simulink model "A63_SwingUp_Control"  (R2022a)
settings: Solver=FixedStepDiscrete  StartTime=0.0  StopTime=inf  FixedStep=0.000125  RelTol=1e-3  EnableMultiTasking=on
PreLoadFcn:
  | RTWConfigurationCB('preloadfcn', bdroot);c2000_ccp_data;
values from neighbouring files (symbols this model uses):
  g = 9.81    [CalcExp.m]    (also in Calculations.m; workspace.mat)
  I = m*l^2/3    (= 0.0027225)    [CalcExp.m]    (also in Calculations.m; workspace.mat)
  K = lqr(A,B,Q,R)    [CalcExp.m]    (also in Calculations.m = lqr(A,B,diag([2000 0 1000 0]),R); rscale.m = k; workspace.mat = [-31.6227766017 -20.1449549457 72.7565036852 9.8125756249])
  l = 0.165    [CalcExp.m]    (also in Calculations.m; experiments.m = P.l*opt.lScale; workspace.mat)
  m = 0.3    [CalcExp.m]    (also in Calculations.m; experiments.m = runAll(makeCtl(c, P), SC, P, opt); workspace.mat)
  Nbar = rscale(sys_ss,K)    [CalcExp.m]    (also in Calculations.m; rscale.m = Nu + K*Nx; workspace.mat = -31.6227766017)
undefined symbols (not defined in the file or in its folder): DiscIntNeverNeededParam, MaxSpeed
libraries: simulink x8, slpidlib x2, lucasnuelle x2
settings Model: SimulationMode=external  ExtModeEnableFloating=off  Creator=The MathWorks, Inc.  LastModifiedBy=Bukarov
settings SolverCC: AlgebraicLoopSolver=TrustRegion
settings DataIOCC: LimitDataPoints=on  SaveFormat=Array  SaveOutput=off  SaveTime=off  ReturnWorkspaceOutputs=off
settings OptimizationCC: DefaultParameterBehavior=Inlined  ExpressionDepthLimit=2147483647  InitFltsAndDblsToZero=on  LifeSpan=inf  MaxStackSize=64  EfficientTunableParamExpr=on
settings DebuggingCC: UnderspecifiedInitializationDetection=Classic  MergeDetectMultiDrivingBlocksExec=none  CheckExecutionContextPreStartOutputMsg=on  SignalResolutionControl=TryResolveAllWithWarning  SolverPrmCheckMsg=warning  MultiTaskDSMMsg=warning  MultiTaskCondExecSysMsg=none  SigSpecEnsureSampleTimeMsg=none  FcnCallInpInsideContextMsg=warning  UnconnectedInputMsg=warning  UnconnectedOutputMsg=warning  UnconnectedLineMsg=warning  AllowSymbolicDim=off  StateNameClashWarn=warning  SFUnexpectedBacktrackingDiag=warning  SFNoUnconditionalDefaultTransitionDiag=warning  SFExecutionAtInitializationDiag=none  SFMachineParentedDataDiag=warning  ArithmeticOperatorsInVariantConditions=warning
settings HardwareCC: ProdBitPerChar=16  ProdBitPerInt=16  ProdBitPerPointer=32  ProdLargestAtomicInteger=Integer  ProdLargestAtomicFloat=None  ProdWordSize=16  ProdHWDeviceType=Texas Instruments->C2000  TargetBitPerChar=16  TargetBitPerInt=16  TargetBitPerPointer=16  TargetLargestAtomicInteger=Integer  TargetIntDivRoundTo=Zero  TargetEndianess=LittleEndian  TargetWordSize=16  TargetHWDeviceType=Texas Instruments->C2000  ProdEqTarget=off
settings ModelReferenceCC: PropagateSignalLabelsOutOfModel=off
settings SFSimCC: SimUseLocalCustomCode=off  SimParseCustomCode=off  MATLABDynamicMemAlloc=off  CustomCodeUndefinedFunction=UseInterfaceOnly
settings RTWCC: SystemTargetFile=ert.tlc  HardwareBoard=TI Delfino F2833x  TemplateMakefile=ert_default_tmf  PostCodeGenCommand=LNPostCodeGenCommand(modelName, buildInfo);codertarget.postCodeGenHookCommand(h)  RTWUseLocalCustomCode=off  CustomInclude="\"C:\\Program Files\\LN\\MatlabToolbox\\lucasnuelle\\codelibs\""  Toolchain=Texas Instruments Code Composer Studio (C2000)  BuildConfiguration=Specify  DLArmComputeVersion=19.05
settings RTWCC: CustomSource=|
  | "C:\Program Files\LN\MatlabToolbox\lucasnuelle\codelibs\sfcn_lnc_wrapper.c"
  | "C:\Program Files\LN\MatlabToolbox\lucasnuelle\codelibs\CO36202A.c"
settings RTWCC: CustomLibrary=|
  | "C:\Program Files\LN\MatlabToolbox\lucasnuelle\codelibs\LNDacCO36202A.lib"
  | "C:\Program Files\LN\MatlabToolbox\lucasnuelle\codelibs\LNComCO36202A.lib"
  | "C:\Program Files\LN\MatlabToolbox\lucasnuelle\codelibs\LNDisplay.lib"
settings CodeAppCC: ForceParamTrailComments=on  IgnoreCustomStorageClasses=off  CustomSymbolStrType=$N$R$M  StateflowObjectComments=on  InternalIdentifier=Classic
settings ERTTargetCC: MultiwordLength=2048  ParMdlRefBuildCompliant=off  CompOptLevelCompliant=off  CPPClassGenCompliant=off  ExtModeStaticAllocSize=2048  ExtModeMexFile=TIC2000ExternalModeOpen  ExtModeIntrfLevel=Level2 - Open  InlinedParameterPlacement=NonHierarchical  ConvertIfToSwitch=off  SuppressUnreachableDefaultCases=off
settings ConfigComp: CovSaveCumulativeToWorkspaceVar=on  CovSaveSingleToWorkspaceVar=on  CovExternalEMLEnable=off  CovSFcnEnable=off

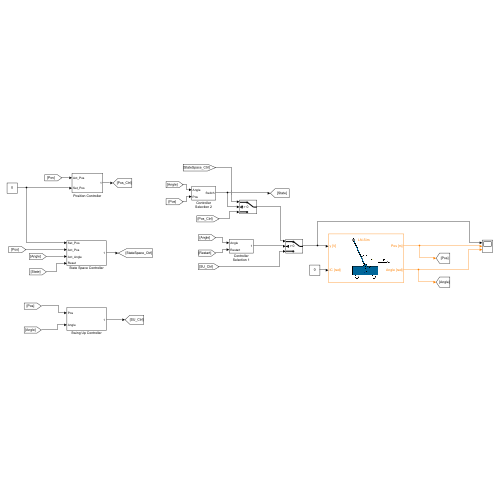
[thumbnail: Simulink's stored preview of the top-level diagram]
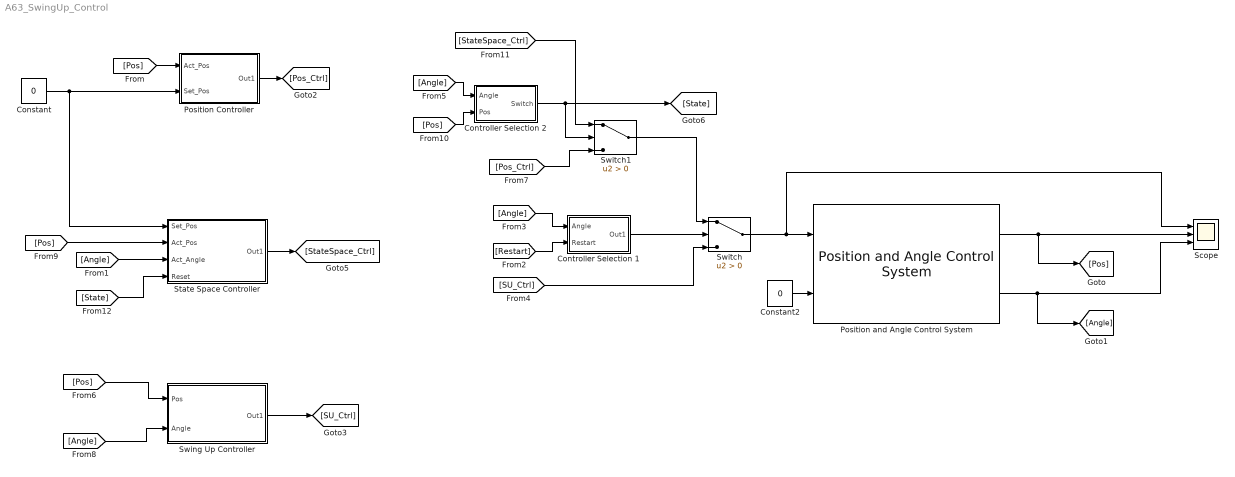
== system A63_SwingUp_Control ==
  Constant : Constant  Value=0
  Constant2 : Constant  Value=0
  Controller Selection 1 : Subsystem
  Controller Selection 2 : Subsystem
  Position Controller : Subsystem
  Position and Angle Control System : lucasnuelle/Simulation/Position and Angle Control System  DefSystem=Predefined  m=0.3  l=0.165  fr=0.3  exportData=on
      settings: SourceProductName=Lucas-Nülle
  Scope : Scope  NumInputPorts=3
  State Space Controller : Subsystem
  Swing Up Controller : Subsystem
  Switch : Switch  Criteria=u2 > Threshold  SaturateOnIntegerOverflow=off  InputSameDT=off
  Switch1 : Switch  Criteria=u2 > Threshold  SaturateOnIntegerOverflow=off  InputSameDT=off
  wires:
  [Angle] -> State Space Controller/3(Act_Angle)
  Constant/1 -> State Space Controller/1(Set_Pos), Position Controller/2(Set_Pos)
  [Pos] -> Position Controller/1(Act_Pos)
  Position Controller/1(Out1) -> [Pos_Ctrl]
  [Pos] -> State Space Controller/2(Act_Pos)
  State Space Controller/1(Out1) -> [StateSpace_Ctrl]
  [State] -> State Space Controller/4(Reset)
  [SU_Ctrl] -> Switch/3
  Controller Selection 1/1(Out1) -> Switch/2
  [Angle] -> Controller Selection 2/1(Angle)
  [Angle] -> Controller Selection 1/1(Angle)
  [Pos] -> Controller Selection 2/2(Pos)
  Switch1/1 -> Switch/1
  [StateSpace_Ctrl] -> Switch1/1
  Controller Selection 2/1(Switch) -> Switch1/2, [State]
  [Pos_Ctrl] -> Switch1/3
  [Restart] -> Controller Selection 1/2(Restart)
  Swing Up Controller/1(Out1) -> [SU_Ctrl]
  [Pos] -> Swing Up Controller/1(Pos)
  [Angle] -> Swing Up Controller/2(Angle)
  Switch/1 -> Scope/1, Position and Angle Control System/1
  Position and Angle Control System/1 -> [Pos], Scope/2
  Position and Angle Control System/2 -> Scope/3, [Angle]
  Constant2/1 -> Position and Angle Control System/2

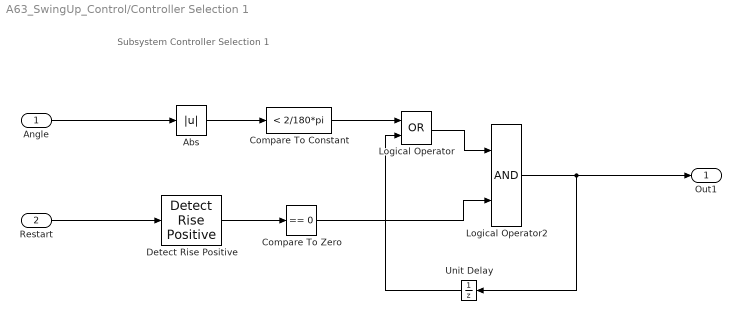
== system A63_SwingUp_Control/Controller Selection 1 ==
  note: Subsystem Controller Selection 1
  Angle : Inport
  Restart : Inport  Port=2
  Abs : Abs  SaturateOnIntegerOverflow=off
  Compare To Constant : simulink/Logic and Bit Operations/Compare To Constant  relop=<  const=2/180*pi  OutDataTypeStr=boolean
  Compare To Zero : simulink/Logic and Bit Operations/Compare To Zero  relop===  OutDataTypeStr=boolean
  Detect Rise Positive : simulink/Logic and Bit Operations/Detect Rise Positive  vinit=0  OutDataTypeStr=boolean
  Logical Operator : Logic  Operator=OR  AllPortsSameDT=off  OutDataTypeStr=boolean
  Logical Operator2 : Logic  AllPortsSameDT=off  OutDataTypeStr=boolean
  Unit Delay : UnitDelay  SampleTime=-1  HasFrameUpgradeWarning=on
  Out1 : Outport
  wires:
  Compare To Zero/1 -> Logical Operator2/2
  Detect Rise Positive/1 -> Compare To Zero/1
  Restart/1 -> Detect Rise Positive/1
  Logical Operator2/1 -> Out1/1, Unit Delay/1
  Compare To Constant/1 -> Logical Operator/1
  Logical Operator/1 -> Logical Operator2/1
  Abs/1 -> Compare To Constant/1
  Angle/1 -> Abs/1
  Unit Delay/1 -> Logical Operator/2

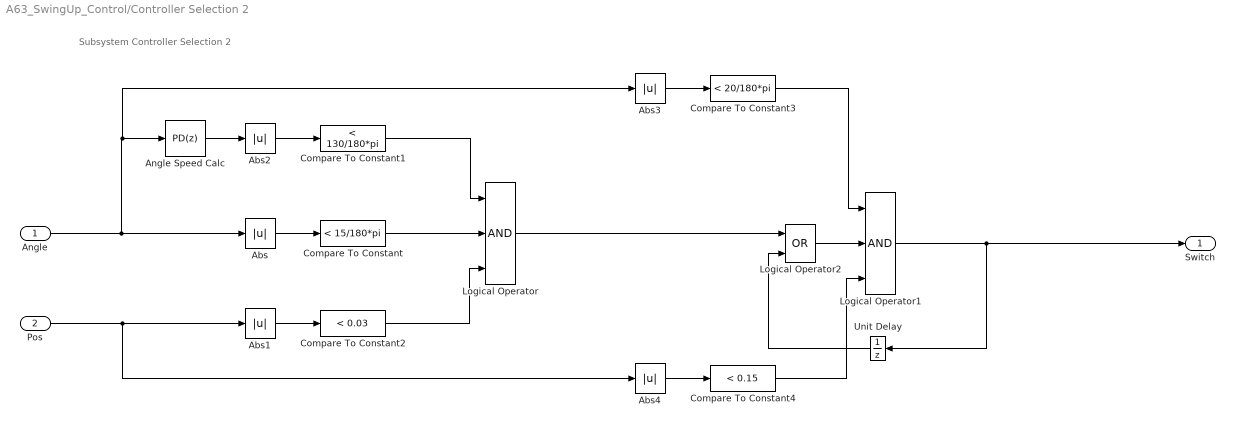
== system A63_SwingUp_Control/Controller Selection 2 ==
  note: Subsystem Controller Selection 2
  Angle : Inport
  Pos : Inport  Port=2
  Abs{,1..4} (5 alike) : Abs  SaturateOnIntegerOverflow=off
  Angle Speed Calc : slpidlib/PID Controller  Controller=PD  Form=Parallel  TimeDomain=Discrete-time  UseExternalTs=off  SampleTime=-1  IntegratorMethod=Forward Euler  FilterMethod=Forward Euler  ControllerParametersSource=internal  P=0  I=1  UseKiTs=off  D=1  N=100  UseFilter=on  TunerSelectOption=Transfer Function Based (PID Tuner App)  InitialConditionSource=internal  InitialConditionForIntegrator=0  InitialConditionForFilter=0  DifferentiatorICPrevScaledInput=0  ExternalReset=none  TrackingMode=off  Kt=1  LimitOutput=off  SatLimitsSource=internal  UpperSaturationLimit=inf  LowerSaturationLimit=-inf  LinearizeAsGain=off  AntiWindupMode=none  Kb=1  POutMin=[]  POutMax=[]  IOutMin=[]  IOutMax=[]  DOutMin=[]  DOutMax=[]  NOutMin=[]  NOutMax=[]  SumOutMin=[]  SumOutMax=[]  SaturationOutMin=[]  SaturationOutMax=[]  PParamMin=[]  PParamMax=[]  IParamMin=[]  IParamMax=[]  DParamMin=[]  DParamMax=[]  NParamMin=[]  NParamMax=[]  KbParamMin=[]  KbParamMax=[]  KtParamMin=[]  KtParamMax=[]  KbOutMin=[]  KbOutMax=[]  KtOutMin=[]  KtOutMax=[]  IntegratorOutMin=[]  IntegratorOutMax=[]  FilterOutMin=[]  FilterOutMax=[]  SumI1OutMin=[]  SumI1OutMax=[]  SumI2OutMin=[]  SumI2OutMax=[]  SumI3OutMin=[]  SumI3OutMax=[]  SumI4OutMin=[]  SumI4OutMax=[]  SumDOutMin=[]  SumDOutMax=[]  DifferentiatorOutMin=[]  DifferentiatorOutMax=[]  FilterDiffOutCoefMin=[]  FilterDiffOutCoefMax=[]  ReciprocalOutMin=[]  ReciprocalOutMax=[]  SumDenOutMin=[]  SumDenOutMax=[]  SumNumOutMin=[]  SumNumOutMax=[]  DivideOutMin=[]  DivideOutMax=[]  UdiffTsProdOutMin=[]  UdiffTsProdOutMax=[]  NTsProdOutMin=[]  NTsProdOutMax=[]  UintegralTsProdOutMin=[]  UintegralTsProdOutMax=[]  UngainTsProdOutMin=[]  UngainTsProdOutMax=[]  IntegratorContinuousStateAttributes=''  IntegratorStateMustResolveToSignalObject=off  IntegratorRTWStateStorageClass=Auto  FilterContinuousStateAttributes=''  FilterStateMustResolveToSignalObject=off  FilterRTWStateStorageClass=Auto  ParallelPVariant=InternalParameters  IdealPVariant=Disabled  IVariant=Disabled  DVariant=InternalParameters  IntegratorVariant=Disabled  SatVariant=Disabled  AWVariant=Disabled  PCopyVariant=Disabled  TRVariant=Disabled  FdbkBlocksVariant=Forward  IdealPFdbkVariant=Disabled  SatFdbkVariant=Disabled  DerivativeFilterVariant=ForwardEulerFilter  NVariant=InternalParameters  NCopyVariant=Disabled  FilterICVariant=InternalICsFilter  IntegratorICVariant=Disabled  ExternalResetVariant=Disabled  TRSumVariant=Passthrough  SumFdbkVariant=Disabled  SumVariant=Sum_PD  TsampFilterVariant=InternalTs  TsampNgainVariant=Passthrough  TsampIntegralVariant=Disabled_SignalSpec  ExternalSaturationOutDataTypeStr=Inherit: Same as second input  aMode=0
  Compare To Constant : simulink/Logic and Bit Operations/Compare To Constant  relop=<  const=15/180*pi  OutDataTypeStr=boolean
  Compare To Constant1 : simulink/Logic and Bit Operations/Compare To Constant  relop=<  const=130/180*pi  OutDataTypeStr=boolean
  Compare To Constant2 : simulink/Logic and Bit Operations/Compare To Constant  relop=<  const=0.03  OutDataTypeStr=boolean
  Compare To Constant3 : simulink/Logic and Bit Operations/Compare To Constant  relop=<  const=20/180*pi  OutDataTypeStr=boolean
  Compare To Constant4 : simulink/Logic and Bit Operations/Compare To Constant  relop=<  const=0.15  OutDataTypeStr=boolean
  Logical Operator : Logic  Inputs=3  AllPortsSameDT=off  OutDataTypeStr=boolean
  Logical Operator1 : Logic  Inputs=3  AllPortsSameDT=off  OutDataTypeStr=boolean
  Logical Operator2 : Logic  Operator=OR  AllPortsSameDT=off  OutDataTypeStr=boolean
  Unit Delay : UnitDelay  SampleTime=-1  HasFrameUpgradeWarning=on
  Switch : Outport
  wires:
  Compare To Constant4/1 -> Logical Operator1/3
  Abs4/1 -> Compare To Constant4/1
  Compare To Constant3/1 -> Logical Operator1/1
  Abs3/1 -> Compare To Constant3/1
  Angle Speed Calc/1 -> Abs2/1
  Compare To Constant1/1 -> Logical Operator/1
  Abs2/1 -> Compare To Constant1/1
  Unit Delay/1 -> Logical Operator2/2
  Logical Operator1/1 -> Switch/1, Unit Delay/1
  Logical Operator2/1 -> Logical Operator1/2
  Compare To Constant2/1 -> Logical Operator/3
  Pos/1 -> Abs1/1, Abs4/1
  Compare To Constant/1 -> Logical Operator/2
  Abs1/1 -> Compare To Constant2/1
  Angle/1 -> Angle Speed Calc/1, Abs3/1, Abs/1
  Abs/1 -> Compare To Constant/1
  Logical Operator/1 -> Logical Operator2/1

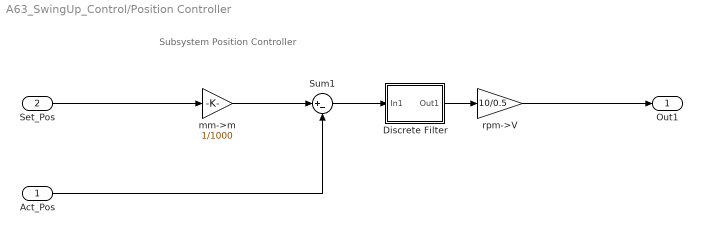
== system A63_SwingUp_Control/Position Controller ==
  note: Subsystem Position Controller
  Act_Pos : Inport
  Set_Pos : Inport  Port=2
  Discrete Filter : Subsystem
  Sum1 : Sum  Inputs=|+-
  mm->m : Gain  Gain=1/1000
  rpm->V : Gain  Gain=10/0.5
  Out1 : Outport
  wires:
  Act_Pos/1 -> Sum1/2
  mm->m/1 -> Sum1/1
  Sum1/1 -> Discrete Filter/1(In1)
  Discrete Filter/1(Out1) -> rpm->V/1
  Set_Pos/1 -> mm->m/1
  rpm->V/1 -> Out1/1

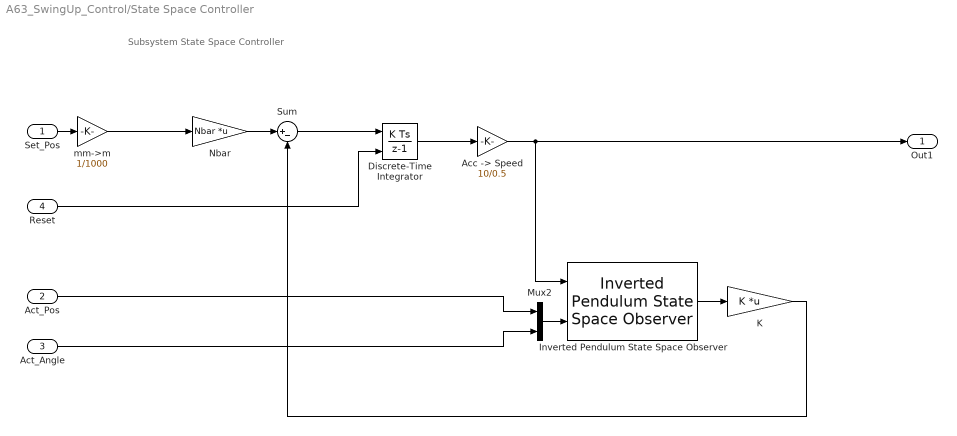
== system A63_SwingUp_Control/State Space Controller ==
  note: Subsystem State Space Controller
  Set_Pos : Inport
  Act_Pos : Inport  Port=2
  Act_Angle : Inport  Port=3
  Reset : Inport  Port=4
  "Acc -> Speed" : Gain  Gain=10/0.5
  Discrete-Time Integrator : DiscreteIntegrator  ExternalReset=rising  SampleTime=-1  ICPrevOutput=DiscIntNeverNeededParam  ICPrevScaledInput=DiscIntNeverNeededParam
  Inverted Pendulum State Space Observer : lucasnuelle/Simulation/Inverted Pendulum State Space Observer  DefSystem=Predefined  m=0.3  l=0.165  fr=0.3  exportData=on
      settings: SourceProductName=Lucas-Nülle
  K : Gain  Gain=K  Multiplication=Matrix(K*u) (u vector)
  Mux2 : Mux  Inputs=2
  Nbar : Gain  Gain=Nbar  Multiplication=Matrix(K*u) (u vector)
  Sum : Sum  Inputs=|+-
  mm->m : Gain  Gain=1/1000
  Out1 : Outport
  wires:
  mm->m/1 -> Nbar/1
  Reset/1 -> Discrete-Time Integrator/2
  Set_Pos/1 -> mm->m/1
  Discrete-Time Integrator/1 -> "Acc -> Speed"/1
  Inverted Pendulum State Space Observer/1 -> K/1
  Nbar/1 -> Sum/1
  Act_Angle/1 -> Mux2/2
  Mux2/1 -> Inverted Pendulum State Space Observer/2
  Sum/1 -> Discrete-Time Integrator/1
  Act_Pos/1 -> Mux2/1
  K/1 -> Sum/2
  "Acc -> Speed"/1 -> Out1/1, Inverted Pendulum State Space Observer/1

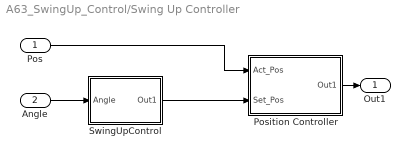
== system A63_SwingUp_Control/Swing Up Controller ==
  Pos : Inport
  Angle : Inport  Port=2
  Position Controller : Subsystem
  SwingUpControl : Subsystem
  Out1 : Outport
  wires:
  Angle/1 -> SwingUpControl/1(Angle)
  Position Controller/1(Out1) -> Out1/1
  SwingUpControl/1(Out1) -> Position Controller/2(Set_Pos)
  Pos/1 -> Position Controller/1(Act_Pos)

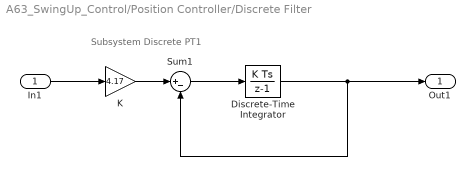
== system A63_SwingUp_Control/Position Controller/Discrete Filter ==
  note: Subsystem Discrete PT1
  In1 : Inport
  Discrete-Time Integrator : DiscreteIntegrator  gainval=1/0.17  SampleTime=-1  ICPrevOutput=DiscIntNeverNeededParam  ICPrevScaledInput=DiscIntNeverNeededParam
  K : Gain  Gain=4.17
  Sum1 : Sum  Inputs=|+-
  Out1 : Outport
  wires:
  Discrete-Time Integrator/1 -> Sum1/2, Out1/1
  K/1 -> Sum1/1
  In1/1 -> K/1
  Sum1/1 -> Discrete-Time Integrator/1

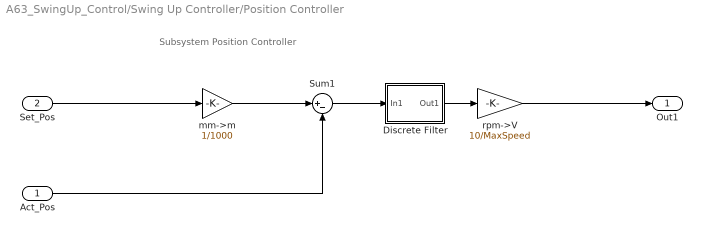
== system A63_SwingUp_Control/Swing Up Controller/Position Controller ==
  note: Subsystem Position Controller
  Act_Pos : Inport
  Set_Pos : Inport  Port=2
  Discrete Filter : Subsystem
  Sum1 : Sum  Inputs=|+-
  mm->m : Gain  Gain=1/1000
  rpm->V : Gain  Gain=10/MaxSpeed
  Out1 : Outport
  wires:
  Act_Pos/1 -> Sum1/2
  mm->m/1 -> Sum1/1
  Sum1/1 -> Discrete Filter/1(In1)
  Discrete Filter/1(Out1) -> rpm->V/1
  Set_Pos/1 -> mm->m/1
  rpm->V/1 -> Out1/1

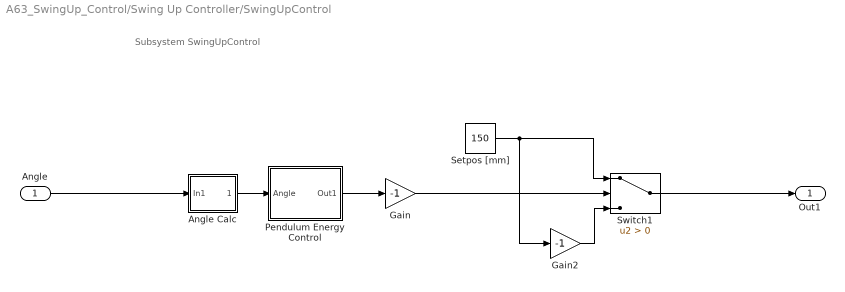
== system A63_SwingUp_Control/Swing Up Controller/SwingUpControl ==
  note: Subsystem SwingUpControl
  Angle : Inport
  Angle Calc : Subsystem
  Gain : Gain  Gain=-1
  Gain2 : Gain  Gain=-1
  Pendulum Energy Control : Subsystem
  Setpos [mm] : Constant  Value=150
  Switch1 : Switch  Criteria=u2 > Threshold  SaturateOnIntegerOverflow=off  InputSameDT=off
  Out1 : Outport
  wires:
  Angle Calc/1(Out1) -> Pendulum Energy Control/1(Angle)
  Gain2/1 -> Switch1/3
  Pendulum Energy Control/1(Out1) -> Gain/1
  Switch1/1 -> Out1/1
  Angle/1 -> Angle Calc/1(In1)
  Gain/1 -> Switch1/2
  Setpos [mm]/1 -> Switch1/1, Gain2/1

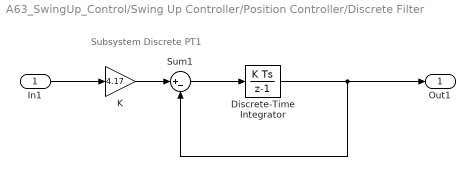
== system A63_SwingUp_Control/Swing Up Controller/Position Controller/Discrete Filter ==
  note: Subsystem Discrete PT1
  In1 : Inport
  Discrete-Time Integrator : DiscreteIntegrator  gainval=1/0.17  SampleTime=-1  ICPrevOutput=DiscIntNeverNeededParam  ICPrevScaledInput=DiscIntNeverNeededParam
  K : Gain  Gain=4.17
  Sum1 : Sum  Inputs=|+-
  Out1 : Outport
  wires:
  Discrete-Time Integrator/1 -> Sum1/2, Out1/1
  K/1 -> Sum1/1
  In1/1 -> K/1
  Sum1/1 -> Discrete-Time Integrator/1

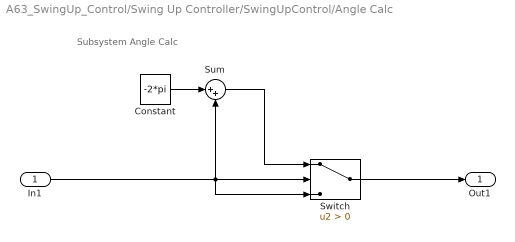
== system A63_SwingUp_Control/Swing Up Controller/SwingUpControl/Angle Calc ==
  note: Subsystem Angle Calc
  In1 : Inport
  Constant : Constant  Value=-2*pi
  Sum : Sum  Inputs=|++
  Switch : Switch  Criteria=u2 > Threshold  SaturateOnIntegerOverflow=off  InputSameDT=off
  Out1 : Outport
  wires:
  Switch/1 -> Out1/1
  In1/1 -> Switch/3, Sum/2, Switch/2
  Constant/1 -> Sum/1
  Sum/1 -> Switch/1

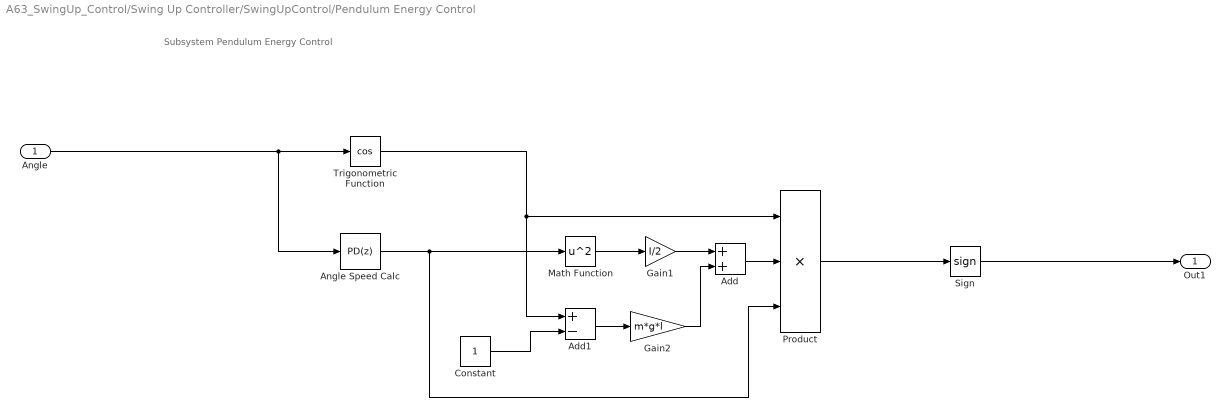
== system A63_SwingUp_Control/Swing Up Controller/SwingUpControl/Pendulum Energy Control ==
  note: Subsystem Pendulum Energy Control
  Angle : Inport
  Add : Sum
  Add1 : Sum  Inputs=+-
  Angle Speed Calc : slpidlib/PID Controller  Controller=PD  Form=Parallel  TimeDomain=Discrete-time  UseExternalTs=off  SampleTime=-1  IntegratorMethod=Forward Euler  FilterMethod=Forward Euler  ControllerParametersSource=internal  P=0  I=1  UseKiTs=off  D=1  N=100  UseFilter=on  TunerSelectOption=Transfer Function Based (PID Tuner App)  InitialConditionSource=internal  InitialConditionForIntegrator=0  InitialConditionForFilter=0  DifferentiatorICPrevScaledInput=0  ExternalReset=none  TrackingMode=off  Kt=1  LimitOutput=off  SatLimitsSource=internal  UpperSaturationLimit=inf  LowerSaturationLimit=-inf  LinearizeAsGain=off  AntiWindupMode=none  Kb=1  POutMin=[]  POutMax=[]  IOutMin=[]  IOutMax=[]  DOutMin=[]  DOutMax=[]  NOutMin=[]  NOutMax=[]  SumOutMin=[]  SumOutMax=[]  SaturationOutMin=[]  SaturationOutMax=[]  PParamMin=[]  PParamMax=[]  IParamMin=[]  IParamMax=[]  DParamMin=[]  DParamMax=[]  NParamMin=[]  NParamMax=[]  KbParamMin=[]  KbParamMax=[]  KtParamMin=[]  KtParamMax=[]  KbOutMin=[]  KbOutMax=[]  KtOutMin=[]  KtOutMax=[]  IntegratorOutMin=[]  IntegratorOutMax=[]  FilterOutMin=[]  FilterOutMax=[]  SumI1OutMin=[]  SumI1OutMax=[]  SumI2OutMin=[]  SumI2OutMax=[]  SumI3OutMin=[]  SumI3OutMax=[]  SumI4OutMin=[]  SumI4OutMax=[]  SumDOutMin=[]  SumDOutMax=[]  DifferentiatorOutMin=[]  DifferentiatorOutMax=[]  FilterDiffOutCoefMin=[]  FilterDiffOutCoefMax=[]  ReciprocalOutMin=[]  ReciprocalOutMax=[]  SumDenOutMin=[]  SumDenOutMax=[]  SumNumOutMin=[]  SumNumOutMax=[]  DivideOutMin=[]  DivideOutMax=[]  UdiffTsProdOutMin=[]  UdiffTsProdOutMax=[]  NTsProdOutMin=[]  NTsProdOutMax=[]  UintegralTsProdOutMin=[]  UintegralTsProdOutMax=[]  UngainTsProdOutMin=[]  UngainTsProdOutMax=[]  IntegratorContinuousStateAttributes=''  IntegratorStateMustResolveToSignalObject=off  IntegratorRTWStateStorageClass=Auto  FilterContinuousStateAttributes=''  FilterStateMustResolveToSignalObject=off  FilterRTWStateStorageClass=Auto  ParallelPVariant=InternalParameters  IdealPVariant=Disabled  IVariant=Disabled  DVariant=InternalParameters  IntegratorVariant=Disabled  SatVariant=Disabled  AWVariant=Disabled  PCopyVariant=Disabled  TRVariant=Disabled  FdbkBlocksVariant=Forward  IdealPFdbkVariant=Disabled  SatFdbkVariant=Disabled  DerivativeFilterVariant=ForwardEulerFilter  NVariant=InternalParameters  NCopyVariant=Disabled  FilterICVariant=InternalICsFilter  IntegratorICVariant=Disabled  ExternalResetVariant=Disabled  TRSumVariant=Passthrough  SumFdbkVariant=Disabled  SumVariant=Sum_PD  TsampFilterVariant=InternalTs  TsampNgainVariant=Passthrough  TsampIntegralVariant=Disabled_SignalSpec  ExternalSaturationOutDataTypeStr=Inherit: Same as second input  aMode=0
  Constant : Constant  SampleTime=-1
  Gain1 : Gain  Gain=I/2
  Gain2 : Gain  Gain=m*g*l
  Math Function : Math  Operator=square  SignedPower=on
  Product : Product  Inputs=3
  Sign : Signum
  Trigonometric Function : Trigonometry  Operator=cos
  Out1 : Outport
  wires:
  Trigonometric Function/1 -> Add1/1, Product/1
  Angle Speed Calc/1 -> Product/3, Math Function/1
  Product/1 -> Sign/1
  Sign/1 -> Out1/1
  Add/1 -> Product/2
  Gain1/1 -> Add/1
  Add1/1 -> Gain2/1
  Gain2/1 -> Add/2
  Constant/1 -> Add1/2
  Angle/1 -> Angle Speed Calc/1, Trigonometric Function/1
  Math Function/1 -> Gain1/1
